simulink model "spray_dryer_fuzzy_pid"  (R2024a)
settings: Solver=ode4  StartTime=0.0  StopTime=P.t_stop  FixedStep=P.dt  RelTol=1e-3
values from neighbouring files (symbols this model uses):
  P = derived(P)    [load_params.m]    (also in regen_fix_figures.m = S.P; run_all_scenarios.m = load_params(); P.sp_spray = sp_spray)
libraries: simulink x11, fuzblock x2
settings Model: Creator=indie  LastModifiedBy=indie
settings DataIOCC: SaveOutput=off  SignalLogging=off  SaveTime=off
settings DebuggingCC: AlgebraicLoopMsg=error  UnconnectedInputMsg=error

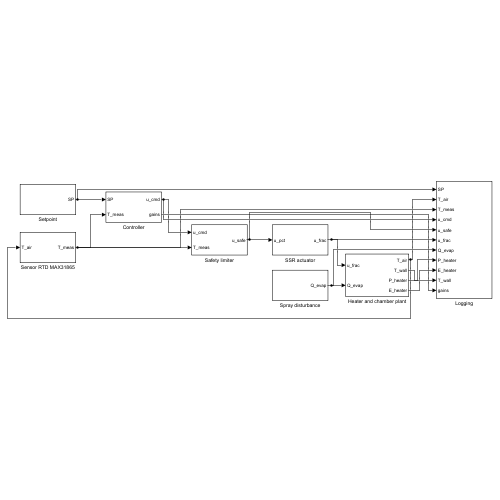
[thumbnail: Simulink's stored preview of the top-level diagram]
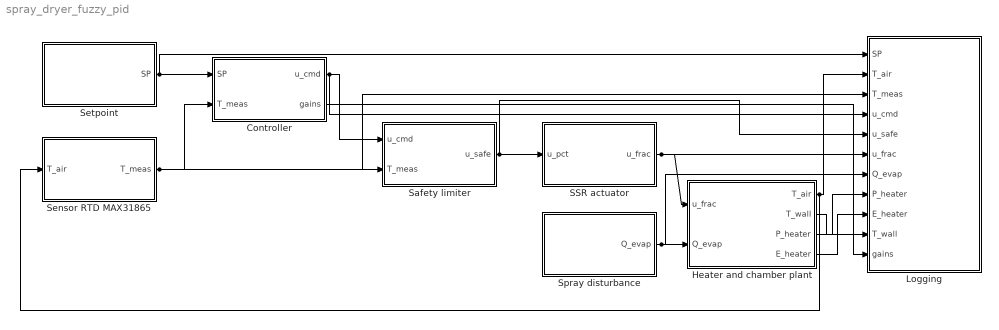
== system spray_dryer_fuzzy_pid ==
  Controller : Subsystem
  Heater and chamber plant : Subsystem
  Logging : Subsystem
  SSR actuator : Subsystem
  Safety limiter : Subsystem
  Sensor RTD MAX31865 : Subsystem
  Setpoint : Subsystem
  Spray disturbance : Subsystem
  wires:
  Controller/2(gains) -> Logging/11(gains)
  Setpoint/1(SP) -> Logging/1(SP), Controller/1(SP)
  Spray disturbance/1(Q_evap) -> Logging/7(Q_evap), Heater and chamber plant/2(Q_evap)
  Sensor RTD MAX31865/1(T_meas) -> Safety limiter/2(T_meas), Logging/3(T_meas), Controller/2(T_meas)
  Heater and chamber plant/1(T_air) -> Sensor RTD MAX31865/1(T_air), Logging/2(T_air)
  Controller/1(u_cmd) -> Logging/4(u_cmd), Safety limiter/1(u_cmd)
  Heater and chamber plant/3(P_heater) -> Logging/8(P_heater)
  Safety limiter/1(u_safe) -> Logging/5(u_safe), SSR actuator/1(u_pct)
  SSR actuator/1(u_frac) -> Logging/6(u_frac), Heater and chamber plant/1(u_frac)
  Heater and chamber plant/2(T_wall) -> Logging/10(T_wall)
  Heater and chamber plant/4(E_heater) -> Logging/9(E_heater)

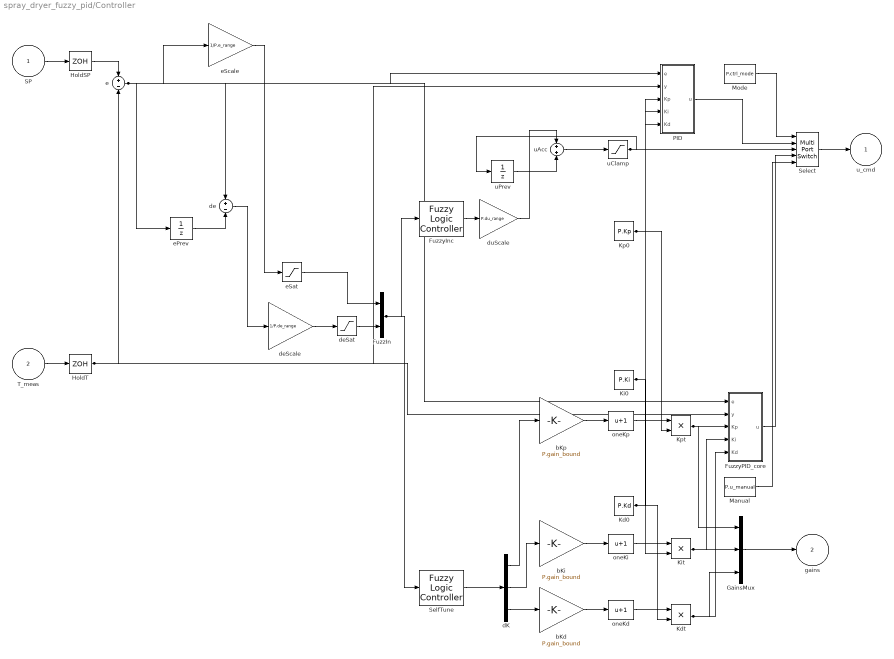
== system spray_dryer_fuzzy_pid/Controller ==
  SP : Inport
  T_meas : Inport  Port=2
  FuzzIn : Mux  Inputs=2
  FuzzyInc : fuzblock/Fuzzy Logic  Controller  FIS=fis_inc  OutputSampleNumber=101  DataType=double  FuzzifiedInputs=off  RuleFiringStrengths=off  RuleOutputs=off  AggregatedOutputs=off  SimulateUsing=Interpreted execution  OutOfRangeInputValueMessage=warning  NoRuleFiredMessage=warning  EmptyOutputFuzzySetMessage=warning
  FuzzyPID_core : Subsystem
  GainsMux : Mux  Inputs=3
  HoldSP : ZeroOrderHold  SampleTime=P.Ts
  HoldT : ZeroOrderHold  SampleTime=P.Ts
  Kd0 : Constant  Value=P.Kd
  Kdt : Product
  Ki0 : Constant  Value=P.Ki
  Kit : Product
  Kp0 : Constant  Value=P.Kp
  Kpt : Product
  Manual : Constant  Value=P.u_manual
  Mode : Constant  Value=P.ctrl_mode
  PID : Subsystem
  Select : MultiPortSwitch  Inputs=4  SaturateOnIntegerOverflow=off  InputSameDT=off
  SelfTune : fuzblock/Fuzzy Logic  Controller  FIS=fis_fpid  OutputSampleNumber=101  DataType=double  FuzzifiedInputs=off  RuleFiringStrengths=off  RuleOutputs=off  AggregatedOutputs=off  SimulateUsing=Interpreted execution  OutOfRangeInputValueMessage=warning  NoRuleFiredMessage=warning  EmptyOutputFuzzySetMessage=warning
  bKd : Gain  Gain=P.gain_bound
  bKi : Gain  Gain=P.gain_bound
  bKp : Gain  Gain=P.gain_bound
  dK : Demux  Outputs=3
  de : Sum  Inputs=+-
  deSat : Saturate  UpperLimit=1  LowerLimit=-1
  deScale : Gain  Gain=1/P.de_range
  duScale : Gain  Gain=P.du_range
  e : Sum  Inputs=+-
  ePrev : UnitDelay  InitialCondition=P.sp_val(1)-P.Tm0  SampleTime=P.Ts  HasFrameUpgradeWarning=on
  eSat : Saturate  UpperLimit=1  LowerLimit=-1
  eScale : Gain  Gain=1/P.e_range
  oneKd : Bias  Bias=1  SaturateOnIntegerOverflow=off
  oneKi : Bias  Bias=1  SaturateOnIntegerOverflow=off
  oneKp : Bias  Bias=1  SaturateOnIntegerOverflow=off
  uAcc : Sum
  uClamp : Saturate  UpperLimit=P.u_max  LowerLimit=P.u_min
  uPrev : UnitDelay  InitialCondition=P.u_min  SampleTime=P.Ts  HasFrameUpgradeWarning=on
  u_cmd : Outport
  gains : Outport  Port=2
  wires:
  SP/1 -> HoldSP/1
  ePrev/1 -> de/2
  T_meas/1 -> HoldT/1
  de/1 -> deScale/1
  HoldSP/1 -> e/1
  HoldT/1 -> e/2, PID/2(y), FuzzyPID_core/2(y)
  e/1 -> eScale/1, FuzzyPID_core/1(e), PID/1(e), ePrev/1, de/1
  eScale/1 -> eSat/1
  eSat/1 -> FuzzIn/1
  Mode/1 -> Select/1
  uAcc/1 -> uClamp/1
  deScale/1 -> deSat/1
  Manual/1 -> Select/5
  bKp/1 -> oneKp/1
  deSat/1 -> FuzzIn/2
  FuzzIn/1 -> FuzzyInc/1, SelfTune/1
  SelfTune/1 -> dK/1
  FuzzyInc/1 -> duScale/1
  oneKp/1 -> Kpt/1
  uPrev/1 -> uAcc/2
  duScale/1 -> uAcc/1
  dK/1 -> bKp/1
  dK/2 -> bKi/1
  dK/3 -> bKd/1
  bKi/1 -> oneKi/1
  bKd/1 -> oneKd/1
  uClamp/1 -> uPrev/1, Select/3
  Kp0/1 -> PID/3(Kp), Kpt/2
  Kit/1 -> GainsMux/2, FuzzyPID_core/4(Ki)
  Ki0/1 -> Kit/2, PID/4(Ki)
  Kd0/1 -> Kdt/2, PID/5(Kd)
  oneKi/1 -> Kit/1
  PID/1(u) -> Select/2
  oneKd/1 -> Kdt/1
  Kpt/1 -> FuzzyPID_core/3(Kp), GainsMux/1
  Kdt/1 -> FuzzyPID_core/5(Kd), GainsMux/3
  FuzzyPID_core/1(u) -> Select/4
  GainsMux/1 -> gains/1
  Select/1 -> u_cmd/1

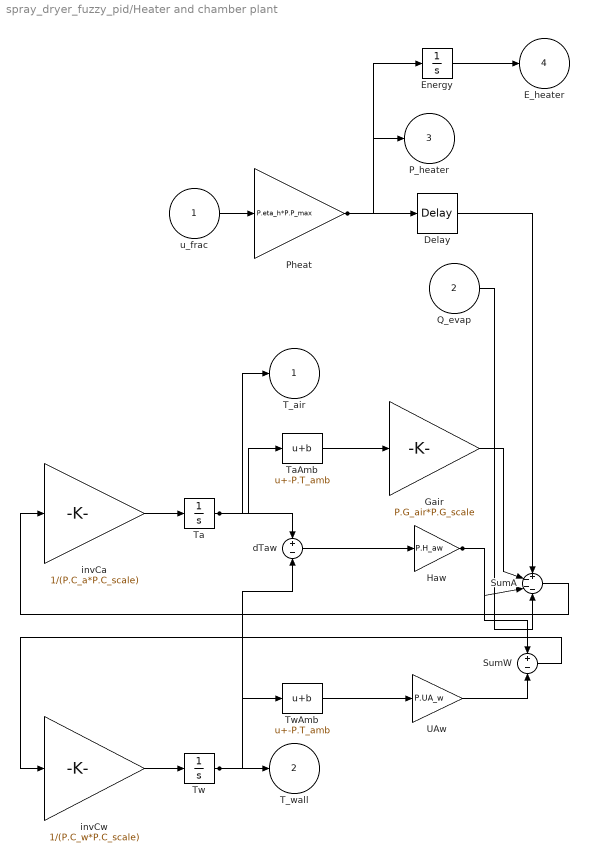
== system spray_dryer_fuzzy_pid/Heater and chamber plant ==
  u_frac : Inport
  Q_evap : Inport  Port=2
  Delay : TransportDelay  DelayTime=P.theta_h+P.theta_extra  InitialOutput=P.eta_h*P.P_max*P.u_init  BufferSize=4096
  Energy : Integrator
  Gair : Gain  Gain=P.G_air*P.G_scale
  Haw : Gain  Gain=P.H_aw
  Pheat : Gain  Gain=P.eta_h*P.P_max
  SumA : Sum  Inputs=+---
  SumW : Sum  Inputs=+-
  Ta : Integrator  InitialCondition=P.Ta0
  TaAmb : Bias  Bias=-P.T_amb  SaturateOnIntegerOverflow=off
  Tw : Integrator  InitialCondition=P.Tw0
  TwAmb : Bias  Bias=-P.T_amb  SaturateOnIntegerOverflow=off
  UAw : Gain  Gain=P.UA_w
  dTaw : Sum  Inputs=+-
  invCa : Gain  Gain=1/(P.C_a*P.C_scale)
  invCw : Gain  Gain=1/(P.C_w*P.C_scale)
  T_air : Outport
  T_wall : Outport  Port=2
  P_heater : Outport  Port=3
  E_heater : Outport  Port=4
  wires:
  u_frac/1 -> Pheat/1
  invCw/1 -> Tw/1
  invCa/1 -> Ta/1
  Tw/1 -> TwAmb/1, T_wall/1, dTaw/2
  Ta/1 -> dTaw/1, TaAmb/1, T_air/1
  Pheat/1 -> Energy/1, Delay/1, P_heater/1
  TaAmb/1 -> Gair/1
  dTaw/1 -> Haw/1
  TwAmb/1 -> UAw/1
  Energy/1 -> E_heater/1
  Delay/1 -> SumA/1
  Q_evap/1 -> SumA/4
  Gair/1 -> SumA/2
  Haw/1 -> SumW/1, SumA/3
  UAw/1 -> SumW/2
  SumA/1 -> invCa/1
  SumW/1 -> invCw/1

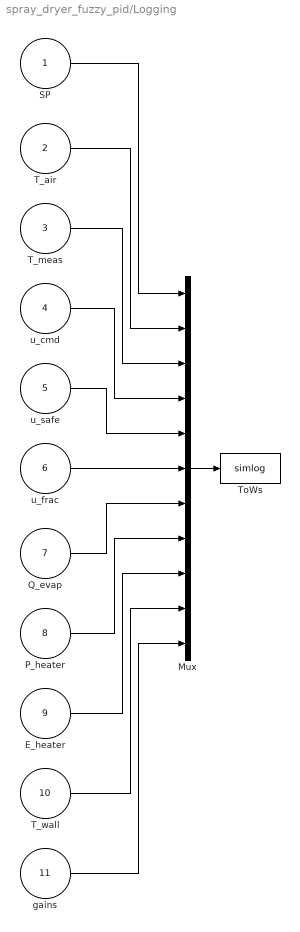
== system spray_dryer_fuzzy_pid/Logging ==
  SP : Inport
  T_air : Inport  Port=2
  T_meas : Inport  Port=3
  u_cmd : Inport  Port=4
  u_safe : Inport  Port=5
  u_frac : Inport  Port=6
  Q_evap : Inport  Port=7
  P_heater : Inport  Port=8
  E_heater : Inport  Port=9
  T_wall : Inport  Port=10
  gains : Inport  Port=11
  Mux : Mux  Inputs=11
  ToWs : ToWorkspace  VariableName=simlog  SaveFormat=Structure With Time  SampleTime=P.log_Ts
  wires:
  SP/1 -> Mux/1
  T_air/1 -> Mux/2
  T_meas/1 -> Mux/3
  u_cmd/1 -> Mux/4
  u_safe/1 -> Mux/5
  u_frac/1 -> Mux/6
  Q_evap/1 -> Mux/7
  P_heater/1 -> Mux/8
  E_heater/1 -> Mux/9
  T_wall/1 -> Mux/10
  gains/1 -> Mux/11
  Mux/1 -> ToWs/1

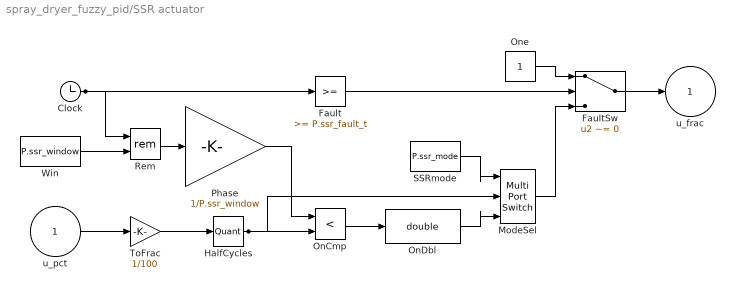
== system spray_dryer_fuzzy_pid/SSR actuator ==
  u_pct : Inport
  Clock : Clock
  Fault : simulink/Logic and Bit Operations/Compare To Constant  relop=>=  const=P.ssr_fault_t  OutDataTypeStr=boolean
  FaultSw : Switch  Criteria=u2 ~= 0  SaturateOnIntegerOverflow=off  InputSameDT=off
  HalfCycles : Quantizer  QuantizationInterval=P.ssr_q
  ModeSel : MultiPortSwitch  Inputs=2  SaturateOnIntegerOverflow=off  InputSameDT=off
  OnCmp : RelationalOperator  Operator=<  OutDataTypeStr=boolean  RndMeth=Simplest  InputSameDT=off
  OnDbl : DataTypeConversion  OutDataTypeStr=double  SaturateOnIntegerOverflow=off  RndMeth=Floor
  One : Constant
  Phase : Gain  Gain=1/P.ssr_window
  Rem : Math  Operator=rem
  SSRmode : Constant  Value=P.ssr_mode
  ToFrac : Gain  Gain=1/100
  Win : Constant  Value=P.ssr_window
  u_frac : Outport
  wires:
  Clock/1 -> Fault/1, Rem/1
  Win/1 -> Rem/2
  u_pct/1 -> ToFrac/1
  Rem/1 -> Phase/1
  ToFrac/1 -> HalfCycles/1
  Phase/1 -> OnCmp/1
  HalfCycles/1 -> ModeSel/2, OnCmp/2
  Fault/1 -> FaultSw/2
  OnCmp/1 -> OnDbl/1
  SSRmode/1 -> ModeSel/1
  OnDbl/1 -> ModeSel/3
  One/1 -> FaultSw/1
  ModeSel/1 -> FaultSw/3
  FaultSw/1 -> u_frac/1

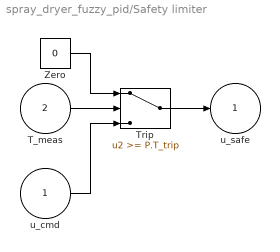
== system spray_dryer_fuzzy_pid/Safety limiter ==
  u_cmd : Inport
  T_meas : Inport  Port=2
  Trip : Switch  Threshold=P.T_trip  SaturateOnIntegerOverflow=off  InputSameDT=off
  Zero : Constant  Value=0
  u_safe : Outport
  wires:
  Zero/1 -> Trip/1
  Trip/1 -> u_safe/1
  T_meas/1 -> Trip/2
  u_cmd/1 -> Trip/3

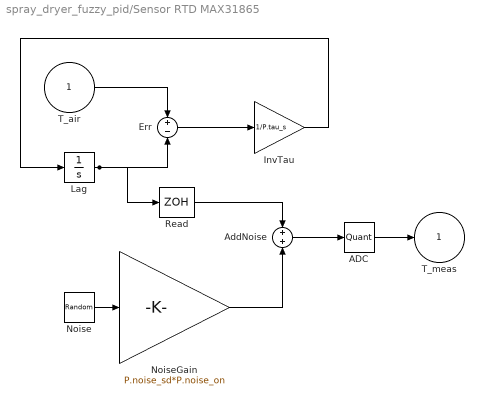
== system spray_dryer_fuzzy_pid/Sensor RTD MAX31865 ==
  T_air : Inport
  ADC : Quantizer  QuantizationInterval=P.adc_q
  AddNoise : Sum
  Err : Sum  Inputs=+-
  InvTau : Gain  Gain=1/P.tau_s
  Lag : Integrator  InitialCondition=P.Tm0
  Noise : RandomNumber  Seed=P.seed  SampleTime=P.Ts_sensor
  NoiseGain : Gain  Gain=P.noise_sd*P.noise_on
  Read : ZeroOrderHold  SampleTime=P.Ts_sensor
  T_meas : Outport
  wires:
  InvTau/1 -> Lag/1
  Noise/1 -> NoiseGain/1
  T_air/1 -> Err/1
  NoiseGain/1 -> AddNoise/2
  Lag/1 -> Err/2, Read/1
  Err/1 -> InvTau/1
  Read/1 -> AddNoise/1
  AddNoise/1 -> ADC/1
  ADC/1 -> T_meas/1

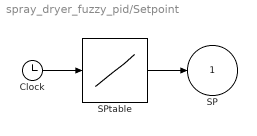
== system spray_dryer_fuzzy_pid/Setpoint ==
  Clock : Clock
  SPtable : Lookup_n-D  NumberOfTableDimensions=1  BreakpointsForDimension1=P.sp_time  Table=P.sp_val  InterpMethod=Flat  ExtrapMethod=Clip  InternalRulePriority=Speed  RndMeth=Simplest
  SP : Outport
  wires:
  Clock/1 -> SPtable/1
  SPtable/1 -> SP/1

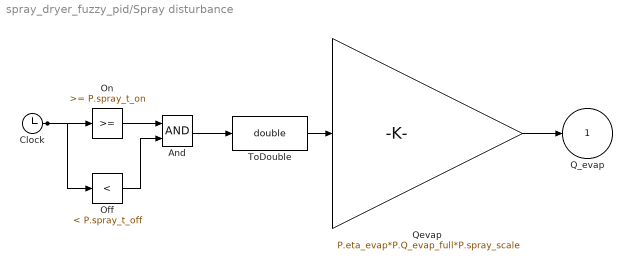
== system spray_dryer_fuzzy_pid/Spray disturbance ==
  And : Logic  AllPortsSameDT=off  OutDataTypeStr=boolean
  Clock : Clock
  Off : simulink/Logic and Bit Operations/Compare To Constant  relop=<  const=P.spray_t_off  OutDataTypeStr=boolean
  On : simulink/Logic and Bit Operations/Compare To Constant  relop=>=  const=P.spray_t_on  OutDataTypeStr=boolean
  Qevap : Gain  Gain=P.eta_evap*P.Q_evap_full*P.spray_scale
  ToDouble : DataTypeConversion  OutDataTypeStr=double  SaturateOnIntegerOverflow=off  RndMeth=Floor
  Q_evap : Outport
  wires:
  Clock/1 -> On/1, Off/1
  Off/1 -> And/2
  On/1 -> And/1
  And/1 -> ToDouble/1
  ToDouble/1 -> Qevap/1
  Qevap/1 -> Q_evap/1

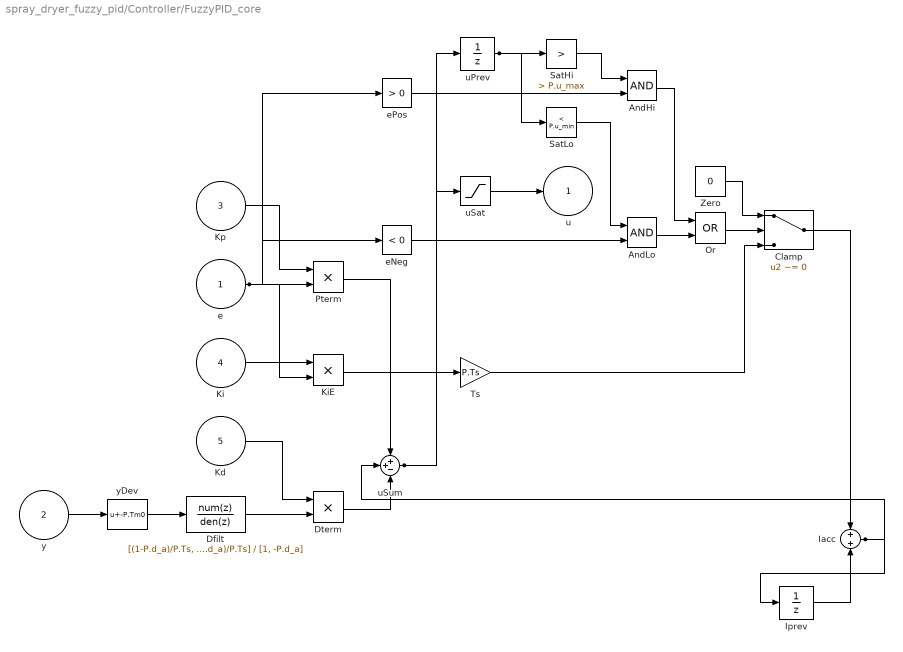
== system spray_dryer_fuzzy_pid/Controller/FuzzyPID_core ==
  e : Inport
  y : Inport  Port=2
  Kp : Inport  Port=3
  Ki : Inport  Port=4
  Kd : Inport  Port=5
  AndHi : Logic  AllPortsSameDT=off  OutDataTypeStr=boolean
  AndLo : Logic  AllPortsSameDT=off  OutDataTypeStr=boolean
  Clamp : Switch  Criteria=u2 ~= 0  SaturateOnIntegerOverflow=off  InputSameDT=off
  Dfilt : DiscreteTransferFcn  Numerator=[(1-P.d_a)/P.Ts, -(1-P.d_a)/P.Ts]  Denominator=[1, -P.d_a]  SampleTime=P.Ts
  Dterm : Product
  Iacc : Sum
  Iprev : UnitDelay  SampleTime=P.Ts  HasFrameUpgradeWarning=on
  KiE : Product
  Or : Logic  Operator=OR  AllPortsSameDT=off  OutDataTypeStr=boolean
  Pterm : Product
  SatHi : simulink/Logic and Bit Operations/Compare To Constant  relop=>  const=P.u_max  OutDataTypeStr=boolean
  SatLo : simulink/Logic and Bit Operations/Compare To Constant  relop=<  const=P.u_min  OutDataTypeStr=boolean
  Ts : Gain  Gain=P.Ts
  Zero : Constant  Value=0
  eNeg : simulink/Logic and Bit Operations/Compare To Zero  relop=<  OutDataTypeStr=boolean
  ePos : simulink/Logic and Bit Operations/Compare To Zero  relop=>  OutDataTypeStr=boolean
  uPrev : UnitDelay  SampleTime=P.Ts  HasFrameUpgradeWarning=on
  uSat : Saturate  UpperLimit=P.u_max  LowerLimit=P.u_min
  uSum : Sum  Inputs=++-
  yDev : Bias  Bias=-P.Tm0  SaturateOnIntegerOverflow=off
  u : Outport
  wires:
  y/1 -> yDev/1
  Pterm/1 -> uSum/1
  Ki/1 -> KiE/1
  uPrev/1 -> SatHi/1, SatLo/1
  yDev/1 -> Dfilt/1
  Kp/1 -> Pterm/1
  Ts/1 -> Clamp/3
  e/1 -> ePos/1, eNeg/1, Pterm/2, KiE/2
  Dfilt/1 -> Dterm/2
  Kd/1 -> Dterm/1
  KiE/1 -> Ts/1
  Dterm/1 -> uSum/3
  ePos/1 -> AndHi/2
  eNeg/1 -> AndLo/2
  uSum/1 -> uPrev/1, uSat/1
  uSat/1 -> u/1
  SatHi/1 -> AndHi/1
  SatLo/1 -> AndLo/1
  AndHi/1 -> Or/1
  AndLo/1 -> Or/2
  Zero/1 -> Clamp/1
  Or/1 -> Clamp/2
  Clamp/1 -> Iacc/1
  Iprev/1 -> Iacc/2
  Iacc/1 -> Iprev/1, uSum/2

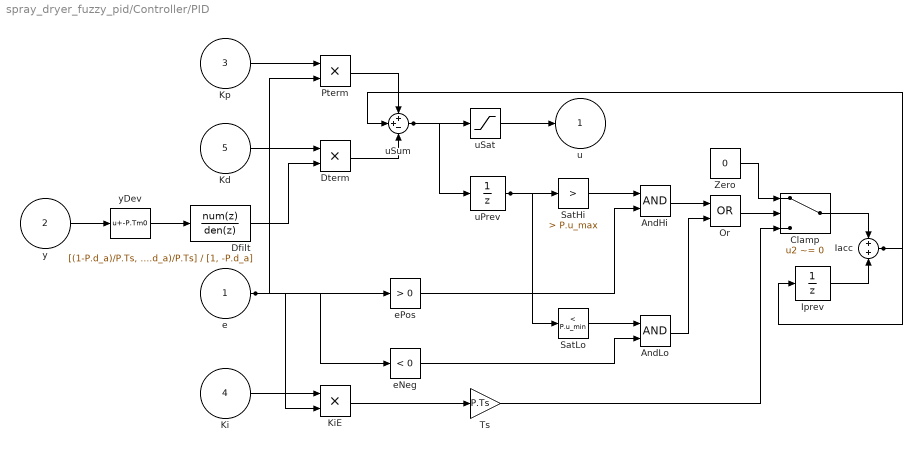
== system spray_dryer_fuzzy_pid/Controller/PID ==
  e : Inport
  y : Inport  Port=2
  Kp : Inport  Port=3
  Ki : Inport  Port=4
  Kd : Inport  Port=5
  AndHi : Logic  AllPortsSameDT=off  OutDataTypeStr=boolean
  AndLo : Logic  AllPortsSameDT=off  OutDataTypeStr=boolean
  Clamp : Switch  Criteria=u2 ~= 0  SaturateOnIntegerOverflow=off  InputSameDT=off
  Dfilt : DiscreteTransferFcn  Numerator=[(1-P.d_a)/P.Ts, -(1-P.d_a)/P.Ts]  Denominator=[1, -P.d_a]  SampleTime=P.Ts
  Dterm : Product
  Iacc : Sum
  Iprev : UnitDelay  SampleTime=P.Ts  HasFrameUpgradeWarning=on
  KiE : Product
  Or : Logic  Operator=OR  AllPortsSameDT=off  OutDataTypeStr=boolean
  Pterm : Product
  SatHi : simulink/Logic and Bit Operations/Compare To Constant  relop=>  const=P.u_max  OutDataTypeStr=boolean
  SatLo : simulink/Logic and Bit Operations/Compare To Constant  relop=<  const=P.u_min  OutDataTypeStr=boolean
  Ts : Gain  Gain=P.Ts
  Zero : Constant  Value=0
  eNeg : simulink/Logic and Bit Operations/Compare To Zero  relop=<  OutDataTypeStr=boolean
  ePos : simulink/Logic and Bit Operations/Compare To Zero  relop=>  OutDataTypeStr=boolean
  uPrev : UnitDelay  SampleTime=P.Ts  HasFrameUpgradeWarning=on
  uSat : Saturate  UpperLimit=P.u_max  LowerLimit=P.u_min
  uSum : Sum  Inputs=++-
  yDev : Bias  Bias=-P.Tm0  SaturateOnIntegerOverflow=off
  u : Outport
  wires:
  y/1 -> yDev/1
  Pterm/1 -> uSum/1
  Ki/1 -> KiE/1
  yDev/1 -> Dfilt/1
  Kp/1 -> Pterm/1
  Dfilt/1 -> Dterm/2
  Kd/1 -> Dterm/1
  AndLo/1 -> Or/2
  e/1 -> ePos/1, KiE/2, Pterm/2, eNeg/1
  Dterm/1 -> uSum/3
  SatLo/1 -> AndLo/1
  KiE/1 -> Ts/1
  uSum/1 -> uPrev/1, uSat/1
  ePos/1 -> AndHi/2
  eNeg/1 -> AndLo/2
  uSat/1 -> u/1
  uPrev/1 -> SatHi/1, SatLo/1
  Ts/1 -> Clamp/3
  SatHi/1 -> AndHi/1
  AndHi/1 -> Or/1
  Zero/1 -> Clamp/1
  Or/1 -> Clamp/2
  Clamp/1 -> Iacc/1
  Iprev/1 -> Iacc/2
  Iacc/1 -> Iprev/1, uSum/2
